simulink model "Comunicacion_arduino_serial_obsevadores_brandon"  (R2021a)
settings: Solver=VariableStepAuto  StartTime=0.0  StopTime=100  RelTol=1e-3
libraries: instrumentseriallib x3
settings Model: Creator=Claudio  LastModifiedBy=ASUS
settings DebuggingCC: UnderspecifiedInitializationDetection=Classic  MergeDetectMultiDrivingBlocksExec=none
settings ModelReferenceCC: PropagateSignalLabelsOutOfModel=off

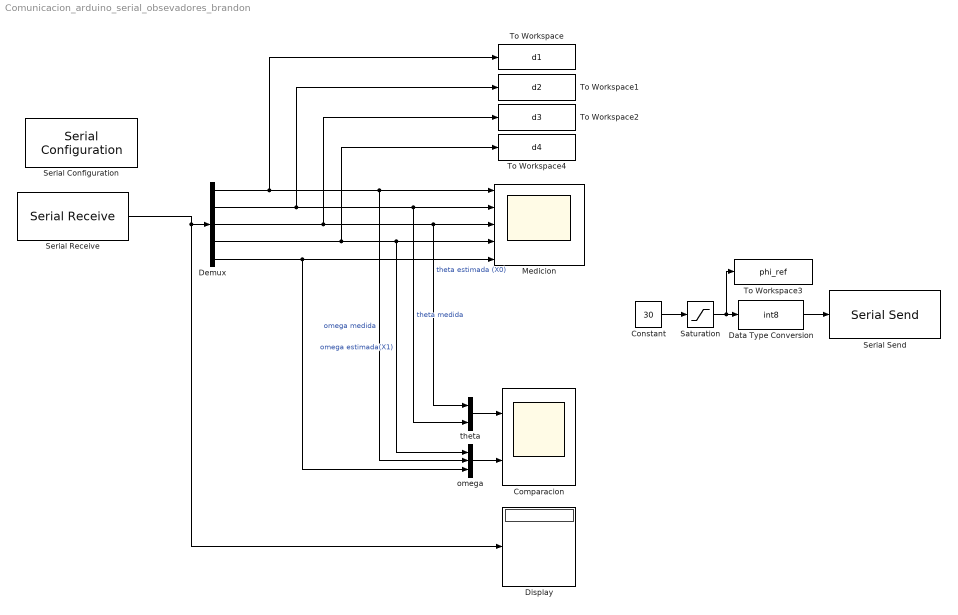
== system Comunicacion_arduino_serial_obsevadores_brandon ==
  Comparacion : Scope  NumInputPorts=2
  Constant : Constant  Value=30
  Data Type Conversion : DataTypeConversion  OutDataTypeStr=int8
  Demux : Demux  Outputs=5
  Display : Display
  Medicion : Scope  NumInputPorts=5
  Saturation : Saturate  UpperLimit=45  LowerLimit=-45
  Serial Configuration : instrumentseriallib/Serial Configuration  Priority=-200000  Port=COM3  ComPort=COM3  BaudRate=115200  DataBits=8  Parity=none  StopBits=1  ByteOrder=little-endian  FlowControl=none  Timeout=10  SimulateUsing=Interpreted execution  BlockInModel=on
  Serial Receive : instrumentseriallib/Serial Receive  Priority=1  Port=COM3  ComPort=COM3  DataType=single  SaveDataType=uint8  ToggleHeader=on  Header="[ 97   98   99  100 ]"  ToggleTerminator=off  Terminator=<none>  CustomTerminator=[]  ToggleDataSize=on  DataSize=[5 1]  EnableBlockingMode=on  ActionDataUnavailable=Output last received value  ActionWhenDataUnavailable=Output last received value  CustomValue=0  SampleTime=0.02  SimulateUsing=Interpreted execution  BlockInModel=on
  Serial Send : instrumentseriallib/Serial Send  Priority=1  Port=COM3  ComPort=COM3  Header=[]  Terminator=<none>  CustomTerminator=[]  EnableBlockingMode=on  SimulateUsing=Interpreted execution  BlockInModel=on
  To Workspace : ToWorkspace  VariableName=d1  SampleTime=-1
      settings: Save2DSignal=2-D array (concatenate along first dimension)
  To Workspace1 : ToWorkspace  VariableName=d2  SampleTime=-1
      settings: Save2DSignal=2-D array (concatenate along first dimension)
  To Workspace2 : ToWorkspace  VariableName=d3  SampleTime=-1
      settings: Save2DSignal=2-D array (concatenate along first dimension)
  To Workspace3 : ToWorkspace  VariableName=phi_ref  SampleTime=0.02
      settings: Save2DSignal=2-D array (concatenate along first dimension)
  To Workspace4 : ToWorkspace  VariableName=d4  SampleTime=-1
      settings: Save2DSignal=2-D array (concatenate along first dimension)
  omega : Mux  Inputs=3
  theta : Mux  Inputs=2
  wires:
  Demux/2 -> To Workspace1/1, theta/2, Medicion/2  "theta medida"
  Demux/1 -> omega/2, Medicion/1, To Workspace/1  "omega medida"
  Demux/3 -> To Workspace2/1, theta/1, Medicion/3  "theta estimada (X0)"
  Constant/1 -> Saturation/1
  Saturation/1 -> To Workspace3/1, Data Type Conversion/1
  Demux/4 -> To Workspace4/1, omega/1, Medicion/4  "omega estimada(X1)"
  theta/1 -> Comparacion/1
  omega/1 -> Comparacion/2
  Serial Receive/1 -> Display/1, Demux/1
  Data Type Conversion/1 -> Serial Send/1
  Demux/5 -> omega/3, Medicion/5
